simulink model "ASM_Traffic"  (R2026a)
settings: Solver=ode1  StartTime=SIM.tstart.v  StopTime=SIM.tend.v  FixedStep=SIM.StepSize.v
PostLoadFcn:
  | if any(exist('dsrtsu_mdlpostloadfcn', 'file') ~= 0), dsrtsu_mdlpostloadfcn('Execute', bdroot); end
  | try, asm_mdl_postloadfcn(bdroot, 'UpdateModel', 3600); catch, disp(lasterr); end,
InitFcn:
  | , if any(exist('rtifpga_mdlclblib', 'file') ~= 0), rtifpga_mdlclblib('Init', bdroot); end,
  | , if any(exist('dsmpb_private', 'file') ~= 0), dsmpb_private('dsmpb_mdlclblib', 'Init', bdroot); end,
model workspace (MAT data in the model file):
  asmReferencePath = [0 0.01 0.02 0.03 0.04 0.05 0.06 0.07 0.08 0.09 0.1 0.11 ... (350007 elements, 50001x7)]
  roadBounds : Simulink.Parameter (value not decoded)
  safetyAxes : Simulink.Parameter (value not decoded)
undefined symbols (not defined in the file): _to_, a0b2, ASM_BrakeHydraulics_DemoSystems, ASM_VehicleDynamics_DemoSystems, b98103fe8ad365046cd0, BrakeCircuit, controllerConfig, CPT, Crankshaft, DiscIntNeverNeededParam, dsmsi, FinalDriveAssembly, MDL, ModeSignals, mu, Pos_BrakePedal_Maneuver, rad, RefSignals, roadFamilyData, roadFamilyId, s_to_rpm, SIM, SoftECU, Suspension, Tire, Transmission
libraries: ASM_Traffic_lib x135, simulink x98, ASM_Utils_lib x77, ASM_VehicleDynamics_lib x70, ASM_Environment_lib x22, dsmpblib x20, dsmsilib x15, MDLD_Utils_lib x10, ASM_BrakeHydraulics_lib x3, sl_discontinuities x2
(part 14 of 65)

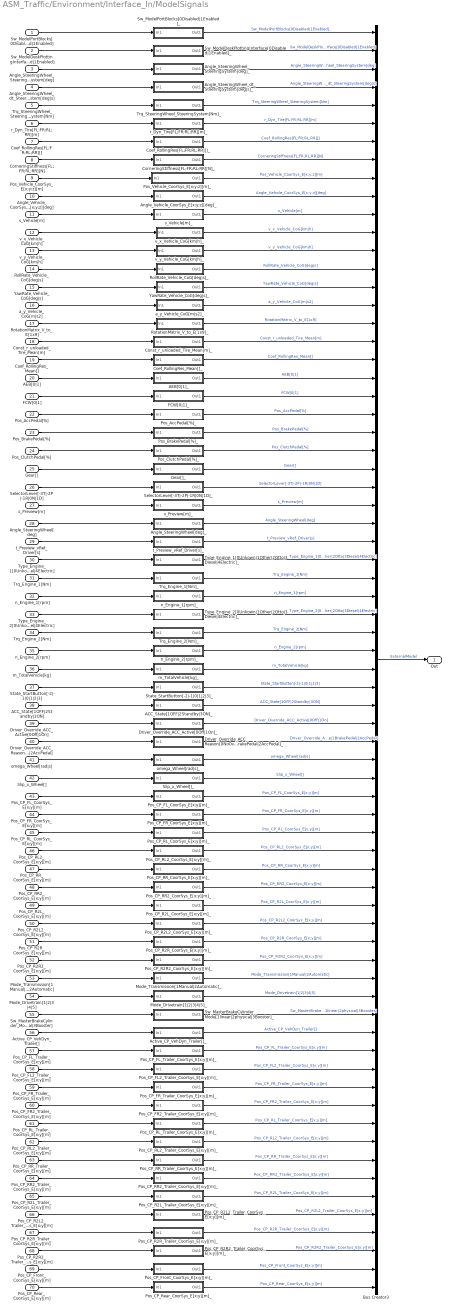
== system ASM_Traffic/Environment/Interface_In/ModelSignals ==
  Sw_ModelPortBlocks[0Disabled|1Enabled] : Inport
  Sw_ModelDeskPlottingInterface[0Disabled|1Enabled] : Inport  Port=2
  Angle_SteeringWheel_SteeringSystem[deg] : Inport  Port=3
  Angle_SteeringWheel_dt_SteeringSystem[deg|s] : Inport  Port=4
  Trq_SteeringWheel_SteeringSystem[Nm] : Inport  Port=5
  r_Dyn_Tire[FL;FR;RL;RR][m] : Inport  Port=6
  Coef_RollingRes[FL;FR;RL;RR][] : Inport  Port=7
  CorneringStiffness[FL;FR;RL;RR][N] : Inport  Port=8
  Pos_Vehicle_CoorSys_E[x;y;z][m] : Inport  Port=9
  Angle_Vehicle_CoorSys_E[x;y;z][deg] : Inport  Port=10
  s_Vehicle[m] : Inport  Port=11
  v_x_Vehicle_CoG[km|h] : Inport  Port=12
  v_y_Vehicle_CoG[km|h] : Inport  Port=13
  RollRate_Vehicle_CoG[deg|s] : Inport  Port=14
  YawRate_Vehicle_CoG[deg|s] : Inport  Port=15
  a_y_Vehicle_CoG[m|s2] : Inport  Port=16
  RotationMatrix_V_to_E[1x9] : Inport  Port=17
  Const_r_unloaded_Tire_Mean[m] : Inport  Port=18
  Coef_RollingRes_Mean[] : Inport  Port=19
  AEB[0|1] : Inport  Port=20
  FCW[0|1] : Inport  Port=21
  Pos_AccPedal[%] : Inport  Port=22
  Pos_BrakePedal[%] : Inport  Port=23
  Pos_ClutchPedal[%] : Inport  Port=24
  Gear[] : Inport  Port=25
  SelectorLever[-3T|-2P|-1R|0N|1D] : Inport  Port=26
  s_Preview[m] : Inport  Port=27
  Angle_SteeringWheel[deg] : Inport  Port=28
  t_Preview_vRef_Driver[s] : Inport  Port=29
  Type_Engine_1[0Unkown|1Other|2Otto|3Diesel|4Electric] : Inport  Port=30
  Trq_Engine_1[Nm] : Inport  Port=31
  n_Engine_1[rpm] : Inport  Port=32
  Type_Engine_2[0Unkown|1Other|2Otto|3Diesel|4Electric] : Inport  Port=33
  Trq_Engine_2[Nm] : Inport  Port=34
  n_Engine_2[rpm] : Inport  Port=35
  m_TotalVehicle[kg] : Inport  Port=36
  State_StartButton[-2|-1|0|1|2|3] : Inport  Port=37
  ACC_State[1OFF|2Standby|3ON] : Inport  Port=38
  Driver_Override_ACC_Active[0Off|1On] : Inport  Port=39
  Driver_Override_ACC_Reason[0NoOverride|1BrakePedal|2AccPedal] : Inport  Port=40
  omega_Wheel[rad|s] : Inport  Port=41
  Slip_x_Wheel[] : Inport  Port=42
  Pos_CP_FL_CoorSys_E[x;y][m] : Inport  Port=43
  Pos_CP_FR_CoorSys_E[x;y][m] : Inport  Port=44
  Pos_CP_RL_CoorSys_E[x;y][m] : Inport  Port=45
  Pos_CP_RL2_CoorSys_E[x;y][m] : Inport  Port=46
  Pos_CP_RR_CoorSys_E[x;y][m] : Inport  Port=47
  Pos_CP_RR2_CoorSys_E[x;y][m] : Inport  Port=48
  Pos_CP_R2L_CoorSys_E[x;y][m] : Inport  Port=49
  Pos_CP_R2L2_CoorSys_E[x;y][m] : Inport  Port=50
  Pos_CP_R2R_CoorSys_E[x;y][m] : Inport  Port=51
  Pos_CP_R2R2_CoorSys_E[x;y][m] : Inport  Port=52
  Mode_Transmission[1Manual|2Automatic] : Inport  Port=53
  Mode_Drivetrain[1|2|3|4|5] : Inport  Port=54
  Sw_MasterBrakeCylinder_Mode[1linear|2physical|3Booster] : Inport  Port=55
  Active_CP_VehDyn_Trailer[] : Inport  Port=56
  Pos_CP_FL_Trailer_CoorSys_E[x;y][m] : Inport  Port=57
  Pos_CP_FL2_Trailer_CoorSys_E[x;y][m] : Inport  Port=58
  Pos_CP_FR_Trailer_CoorSys_E[x;y][m] : Inport  Port=59
  Pos_CP_FR2_Trailer_CoorSys_E[x;y][m] : Inport  Port=60
  Pos_CP_RL_Trailer_CoorSys_E[x;y][m] : Inport  Port=61
  Pos_CP_RL2_Trailer_CoorSys_E[x;y][m] : Inport  Port=62
  Pos_CP_RR_Trailer_CoorSys_E[x;y][m] : Inport  Port=63
  Pos_CP_RR2_Trailer_CoorSys_E[x;y][m] : Inport  Port=64
  Pos_CP_R2L_Trailer_CoorSys_E[x;y][m] : Inport  Port=65
  Pos_CP_R2L2_Trailer_CoorSys_E[x;y][m] : Inport  Port=66
  Pos_CP_R2R_Trailer_CoorSys_E[x;y][m] : Inport  Port=67
  Pos_CP_R2R2_Trailer_CoorSys_E[x;y][m] : Inport  Port=68
  Pos_CP_Front_CoorSys_E[x;y][m] : Inport  Port=69
  Pos_CP_Rear_CoorSys_E[x;y][m] : Inport  Port=70
  ACC_State[1OFF|2Standby|3ON]_ : Subsystem
      mask Display: disp('')
  AEB[0|1]_ : Subsystem
      mask Display: disp('')
  Active_CP_VehDyn_Trailer[]_ : Subsystem
      mask Display: disp('')
  Angle_SteeringWheel[deg]_ : Subsystem
      mask Display: disp('')
  Angle_SteeringWheel_SteeringSystem[deg]_ : Subsystem
      mask Display: disp('')
  Angle_SteeringWheel_dt_SteeringSystem[deg|s]_ : Subsystem
      mask Display: disp('')
  Angle_Vehicle_CoorSys_E[x;y;z][deg]_ : Subsystem
      mask Display: disp('')
  Bus Creator3 : BusCreator  Inputs=70
  Coef_RollingRes[FL;FR;RL;RR][]_ : Subsystem
      mask Display: disp('')
  Coef_RollingRes_Mean[]_ : Subsystem
      mask Display: disp('')
  Const_r_unloaded_Tire_Mean[m]_ : Subsystem
      mask Display: disp('')
  CorneringStiffness[FL;FR;RL;RR][N]_ : Subsystem
      mask Display: disp('')
  Driver_Override_ACC_Active[0Off|1On]_ : Subsystem
      mask Display: disp('')
  Driver_Override_ACC_Reason[0NoOverride|1BrakePedal|2AccPedal]_ : Subsystem
      mask Display: disp('')
  FCW[0|1]_ : Subsystem
      mask Display: disp('')
  Gear[]_ : Subsystem
      mask Display: disp('')
  Mode_Drivetrain[1|2|3|4|5]_ : Subsystem
      mask Display: disp('')
  Mode_Transmission[1Manual|2Automatic]_ : Subsystem
      mask Display: disp('')
  Pos_AccPedal[%]_ : Subsystem
      mask Display: disp('')
  Pos_BrakePedal[%]_ : Subsystem
      mask Display: disp('')
  Pos_CP_FL2_Trailer_CoorSys_E[x;y][m]_ : Subsystem
      mask Display: disp('')
  Pos_CP_FL_CoorSys_E[x;y][m]_ : Subsystem
      mask Display: disp('')
  Pos_CP_FL_Trailer_CoorSys_E[x;y][m]_ : Subsystem
      mask Display: disp('')
  Pos_CP_FR2_Trailer_CoorSys_E[x;y][m]_ : Subsystem
      mask Display: disp('')
  Pos_CP_FR_CoorSys_E[x;y][m]_ : Subsystem
      mask Display: disp('')
  Pos_CP_FR_Trailer_CoorSys_E[x;y][m]_ : Subsystem
      mask Display: disp('')
  Pos_CP_Front_CoorSys_E[x;y][m]_ : Subsystem
      mask Display: disp('')
  Pos_CP_R2L2_CoorSys_E[x;y][m]_ : Subsystem
      mask Display: disp('')
  Pos_CP_R2L2_Trailer_CoorSys_E[x;y][m]_ : Subsystem
      mask Display: disp('')
  Pos_CP_R2L_CoorSys_E[x;y][m]_ : Subsystem
      mask Display: disp('')
  Pos_CP_R2L_Trailer_CoorSys_E[x;y][m]_ : Subsystem
      mask Display: disp('')
  Pos_CP_R2R2_CoorSys_E[x;y][m]_ : Subsystem
      mask Display: disp('')
  Pos_CP_R2R2_Trailer_CoorSys_E[x;y][m]_ : Subsystem
      mask Display: disp('')
  Pos_CP_R2R_CoorSys_E[x;y][m]_ : Subsystem
      mask Display: disp('')
  Pos_CP_R2R_Trailer_CoorSys_E[x;y][m]_ : Subsystem
      mask Display: disp('')
  Pos_CP_RL2_CoorSys_E[x;y][m]_ : Subsystem
      mask Display: disp('')
  Pos_CP_RL2_Trailer_CoorSys_E[x;y][m]_ : Subsystem
      mask Display: disp('')
  Pos_CP_RL_CoorSys_E[x;y][m]_ : Subsystem
      mask Display: disp('')
  Pos_CP_RL_Trailer_CoorSys_E[x;y][m]_ : Subsystem
      mask Display: disp('')
  Pos_CP_RR2_CoorSys_E[x;y][m]_ : Subsystem
      mask Display: disp('')
  Pos_CP_RR2_Trailer_CoorSys_E[x;y][m]_ : Subsystem
      mask Display: disp('')
  Pos_CP_RR_CoorSys_E[x;y][m]_ : Subsystem
      mask Display: disp('')
  Pos_CP_RR_Trailer_CoorSys_E[x;y][m]_ : Subsystem
      mask Display: disp('')
  Pos_CP_Rear_CoorSys_E[x;y][m]_ : Subsystem
      mask Display: disp('')
  Pos_ClutchPedal[%]_ : Subsystem
      mask Display: disp('')
  Pos_Vehicle_CoorSys_E[x;y;z][m]_ : Subsystem
      mask Display: disp('')
  RollRate_Vehicle_CoG[deg|s]_ : Subsystem
      mask Display: disp('')
  RotationMatrix_V_to_E[1x9]_ : Subsystem
      mask Display: disp('')
  SelectorLever[-3T|-2P|-1R|0N|1D]_ : Subsystem
      mask Display: disp('')
  Slip_x_Wheel[]_ : Subsystem
      mask Display: disp('')
  State_StartButton[-2|-1|0|1|2|3]_ : Subsystem
      mask Display: disp('')
  Sw_MasterBrakeCylinder_Mode[1linear|2physical|3Booster]_ : Subsystem
      mask Display: disp('')
  Sw_ModelDeskPlottingInterface[0Disabled|1Enabled]_ : Subsystem
  Sw_ModelPortBlocks[0Disabled|1Enabled]_ : Subsystem
  Trq_Engine_1[Nm]_ : Subsystem
      mask Display: disp('')
  Trq_Engine_2[Nm]_ : Subsystem
      mask Display: disp('')
  Trq_SteeringWheel_SteeringSystem[Nm]_ : Subsystem
      mask Display: disp('')
  Type_Engine_1[0Unkown|1Other|2Otto|3Diesel|4Electric]_ : Subsystem
      mask Display: disp('')
  Type_Engine_2[0Unkown|1Other|2Otto|3Diesel|4Electric]_ : Subsystem
      mask Display: disp('')
  YawRate_Vehicle_CoG[deg|s]_ : Subsystem
      mask Display: disp('')
  a_y_Vehicle_CoG[m|s2]_ : Subsystem
      mask Display: disp('')
  m_TotalVehicle[kg]_ : Subsystem
      mask Display: disp('')
  n_Engine_1[rpm]_ : Subsystem
      mask Display: disp('')
  n_Engine_2[rpm]_ : Subsystem
      mask Display: disp('')
  omega_Wheel[rad|s]_ : Subsystem
      mask Display: disp('')
  r_Dyn_Tire[FL;FR;RL;RR][m]_ : Subsystem
      mask Display: disp('')
  s_Preview[m]_ : Subsystem
      mask Display: disp('')
  s_Vehicle[m]_ : Subsystem
      mask Display: disp('')
  t_Preview_vRef_Driver[s]_ : Subsystem
      mask Display: disp('')
  v_x_Vehicle_CoG[km|h]_ : Subsystem
      mask Display: disp('')
  v_y_Vehicle_CoG[km|h]_ : Subsystem
      mask Display: disp('')
  Out : Outport  VectorParamsAs1DForOutWhenUnconnected=off
  wires:
  Pos_CP_Front_CoorSys_E[x;y][m]/1 -> Pos_CP_Front_CoorSys_E[x;y][m]_/1(In1)
  Pos_CP_Rear_CoorSys_E[x;y][m]_/1(Out1) -> Bus Creator3/70  "Pos_CP_Rear_CoorSys_E[x;y][m]"
  Pos_CP_Rear_CoorSys_E[x;y][m]/1 -> Pos_CP_Rear_CoorSys_E[x;y][m]_/1(In1)
  Pos_CP_Front_CoorSys_E[x;y][m]_/1(Out1) -> Bus Creator3/69  "Pos_CP_Front_CoorSys_E[x;y][m]"
  Sw_ModelDeskPlottingInterface[0Disabled|1Enabled]_/1(Out1) -> Bus Creator3/2  "Sw_ModelDeskPlottingInterface[0Disabled|1Enabled]"
  Sw_ModelPortBlocks[0Disabled|1Enabled]_/1(Out1) -> Bus Creator3/1  "Sw_ModelPortBlocks[0Disabled|1Enabled]"
  Sw_ModelDeskPlottingInterface[0Disabled|1Enabled]/1 -> Sw_ModelDeskPlottingInterface[0Disabled|1Enabled]_/1(In1)
  Sw_ModelPortBlocks[0Disabled|1Enabled]/1 -> Sw_ModelPortBlocks[0Disabled|1Enabled]_/1(In1)
  Bus Creator3/1 -> Out/1  "ExternalModel"
  Trq_SteeringWheel_SteeringSystem[Nm]/1 -> Trq_SteeringWheel_SteeringSystem[Nm]_/1(In1)
  Angle_SteeringWheel_SteeringSystem[deg]/1 -> Angle_SteeringWheel_SteeringSystem[deg]_/1(In1)
  Angle_SteeringWheel_SteeringSystem[deg]_/1(Out1) -> Bus Creator3/3  "Angle_SteeringWheel_SteeringSystem[deg]"
  Trq_SteeringWheel_SteeringSystem[Nm]_/1(Out1) -> Bus Creator3/5  "Trq_SteeringWheel_SteeringSystem[Nm]"
  Pos_CP_RR2_CoorSys_E[x;y][m]_/1(Out1) -> Bus Creator3/48  "Pos_CP_RR2_CoorSys_E[x;y][m]"
  Coef_RollingRes[FL;FR;RL;RR][]_/1(Out1) -> Bus Creator3/7  "Coef_RollingRes[FL;FR;RL;RR][]"
  Coef_RollingRes_Mean[]_/1(Out1) -> Bus Creator3/19  "Coef_RollingRes_Mean[]"
  Active_CP_VehDyn_Trailer[]_/1(Out1) -> Bus Creator3/56  "Active_CP_VehDyn_Trailer[]"
  Pos_CP_RR_Trailer_CoorSys_E[x;y][m]_/1(Out1) -> Bus Creator3/63  "Pos_CP_RR_Trailer_CoorSys_E[x;y][m]"
  Pos_CP_FL_Trailer_CoorSys_E[x;y][m]_/1(Out1) -> Bus Creator3/57  "Pos_CP_FL_Trailer_CoorSys_E[x;y][m]"
  Pos_CP_R2R_CoorSys_E[x;y][m]_/1(Out1) -> Bus Creator3/51  "Pos_CP_R2R_CoorSys_E[x;y][m]"
  Pos_CP_R2R2_Trailer_CoorSys_E[x;y][m]_/1(Out1) -> Bus Creator3/68  "Pos_CP_R2R2_Trailer_CoorSys_E[x;y][m]"
  Pos_CP_R2L_Trailer_CoorSys_E[x;y][m]_/1(Out1) -> Bus Creator3/65  "Pos_CP_R2L_Trailer_CoorSys_E[x;y][m]"
  Pos_CP_FR_CoorSys_E[x;y][m]_/1(Out1) -> Bus Creator3/44  "Pos_CP_FR_CoorSys_E[x;y][m]"
  Pos_CP_FR_Trailer_CoorSys_E[x;y][m]_/1(Out1) -> Bus Creator3/59  "Pos_CP_FR_Trailer_CoorSys_E[x;y][m]"
  Pos_CP_R2L2_Trailer_CoorSys_E[x;y][m]_/1(Out1) -> Bus Creator3/66  "Pos_CP_R2L2_Trailer_CoorSys_E[x;y][m]"
  Pos_CP_R2L2_CoorSys_E[x;y][m]_/1(Out1) -> Bus Creator3/50  "Pos_CP_R2L2_CoorSys_E[x;y][m]"
  Pos_CP_RL_Trailer_CoorSys_E[x;y][m]_/1(Out1) -> Bus Creator3/61  "Pos_CP_RL_Trailer_CoorSys_E[x;y][m]"
  Pos_CP_RL_CoorSys_E[x;y][m]_/1(Out1) -> Bus Creator3/45  "Pos_CP_RL_CoorSys_E[x;y][m]"
  Pos_CP_RR2_Trailer_CoorSys_E[x;y][m]_/1(Out1) -> Bus Creator3/64  "Pos_CP_RR2_Trailer_CoorSys_E[x;y][m]"
  r_Dyn_Tire[FL;FR;RL;RR][m]_/1(Out1) -> Bus Creator3/6  "r_Dyn_Tire[FL;FR;RL;RR][m]"
  Pos_CP_R2R2_CoorSys_E[x;y][m]_/1(Out1) -> Bus Creator3/52  "Pos_CP_R2R2_CoorSys_E[x;y][m]"
  Pos_CP_RR_CoorSys_E[x;y][m]_/1(Out1) -> Bus Creator3/47  "Pos_CP_RR_CoorSys_E[x;y][m]"
  Const_r_unloaded_Tire_Mean[m]_/1(Out1) -> Bus Creator3/18  "Const_r_unloaded_Tire_Mean[m]"
  Pos_CP_FR2_Trailer_CoorSys_E[x;y][m]_/1(Out1) -> Bus Creator3/60  "Pos_CP_FR2_Trailer_CoorSys_E[x;y][m]"
  Pos_CP_RL2_CoorSys_E[x;y][m]_/1(Out1) -> Bus Creator3/46  "Pos_CP_RL2_CoorSys_E[x;y][m]"
  Pos_CP_FL_CoorSys_E[x;y][m]_/1(Out1) -> Bus Creator3/43  "Pos_CP_FL_CoorSys_E[x;y][m]"
  Pos_CP_FL2_Trailer_CoorSys_E[x;y][m]_/1(Out1) -> Bus Creator3/58  "Pos_CP_FL2_Trailer_CoorSys_E[x;y][m]"
  Pos_CP_RL2_Trailer_CoorSys_E[x;y][m]_/1(Out1) -> Bus Creator3/62  "Pos_CP_RL2_Trailer_CoorSys_E[x;y][m]"
  Pos_CP_R2R_Trailer_CoorSys_E[x;y][m]_/1(Out1) -> Bus Creator3/67  "Pos_CP_R2R_Trailer_CoorSys_E[x;y][m]"
  Pos_CP_R2L_CoorSys_E[x;y][m]_/1(Out1) -> Bus Creator3/49  "Pos_CP_R2L_CoorSys_E[x;y][m]"
  CorneringStiffness[FL;FR;RL;RR][N]_/1(Out1) -> Bus Creator3/8  "CorneringStiffness[FL;FR;RL;RR][N]"
  r_Dyn_Tire[FL;FR;RL;RR][m]/1 -> r_Dyn_Tire[FL;FR;RL;RR][m]_/1(In1)
  Const_r_unloaded_Tire_Mean[m]/1 -> Const_r_unloaded_Tire_Mean[m]_/1(In1)
  Coef_RollingRes[FL;FR;RL;RR][]/1 -> Coef_RollingRes[FL;FR;RL;RR][]_/1(In1)
  Coef_RollingRes_Mean[]/1 -> Coef_RollingRes_Mean[]_/1(In1)
  CorneringStiffness[FL;FR;RL;RR][N]/1 -> CorneringStiffness[FL;FR;RL;RR][N]_/1(In1)
  Pos_CP_FL_CoorSys_E[x;y][m]/1 -> Pos_CP_FL_CoorSys_E[x;y][m]_/1(In1)
  Pos_CP_FR_CoorSys_E[x;y][m]/1 -> Pos_CP_FR_CoorSys_E[x;y][m]_/1(In1)
  Pos_CP_RL_CoorSys_E[x;y][m]/1 -> Pos_CP_RL_CoorSys_E[x;y][m]_/1(In1)
  Pos_CP_RL2_CoorSys_E[x;y][m]/1 -> Pos_CP_RL2_CoorSys_E[x;y][m]_/1(In1)
  Pos_CP_RR_CoorSys_E[x;y][m]/1 -> Pos_CP_RR_CoorSys_E[x;y][m]_/1(In1)
  Pos_CP_RR2_CoorSys_E[x;y][m]/1 -> Pos_CP_RR2_CoorSys_E[x;y][m]_/1(In1)
  Pos_CP_R2L_CoorSys_E[x;y][m]/1 -> Pos_CP_R2L_CoorSys_E[x;y][m]_/1(In1)
  Pos_CP_R2L2_CoorSys_E[x;y][m]/1 -> Pos_CP_R2L2_CoorSys_E[x;y][m]_/1(In1)
  Pos_CP_R2R_CoorSys_E[x;y][m]/1 -> Pos_CP_R2R_CoorSys_E[x;y][m]_/1(In1)
  Pos_CP_R2R2_CoorSys_E[x;y][m]/1 -> Pos_CP_R2R2_CoorSys_E[x;y][m]_/1(In1)
  Pos_CP_FL_Trailer_CoorSys_E[x;y][m]/1 -> Pos_CP_FL_Trailer_CoorSys_E[x;y][m]_/1(In1)
  Pos_CP_FL2_Trailer_CoorSys_E[x;y][m]/1 -> Pos_CP_FL2_Trailer_CoorSys_E[x;y][m]_/1(In1)
  Pos_CP_FR_Trailer_CoorSys_E[x;y][m]/1 -> Pos_CP_FR_Trailer_CoorSys_E[x;y][m]_/1(In1)
  Pos_CP_FR2_Trailer_CoorSys_E[x;y][m]/1 -> Pos_CP_FR2_Trailer_CoorSys_E[x;y][m]_/1(In1)
  Pos_CP_RL_Trailer_CoorSys_E[x;y][m]/1 -> Pos_CP_RL_Trailer_CoorSys_E[x;y][m]_/1(In1)
  Pos_CP_RL2_Trailer_CoorSys_E[x;y][m]/1 -> Pos_CP_RL2_Trailer_CoorSys_E[x;y][m]_/1(In1)
  Pos_CP_RR_Trailer_CoorSys_E[x;y][m]/1 -> Pos_CP_RR_Trailer_CoorSys_E[x;y][m]_/1(In1)
  Pos_CP_RR2_Trailer_CoorSys_E[x;y][m]/1 -> Pos_CP_RR2_Trailer_CoorSys_E[x;y][m]_/1(In1)
  Pos_CP_R2L_Trailer_CoorSys_E[x;y][m]/1 -> Pos_CP_R2L_Trailer_CoorSys_E[x;y][m]_/1(In1)
  Pos_CP_R2L2_Trailer_CoorSys_E[x;y][m]/1 -> Pos_CP_R2L2_Trailer_CoorSys_E[x;y][m]_/1(In1)
  Pos_CP_R2R_Trailer_CoorSys_E[x;y][m]/1 -> Pos_CP_R2R_Trailer_CoorSys_E[x;y][m]_/1(In1)
  Pos_CP_R2R2_Trailer_CoorSys_E[x;y][m]/1 -> Pos_CP_R2R2_Trailer_CoorSys_E[x;y][m]_/1(In1)
  Active_CP_VehDyn_Trailer[]/1 -> Active_CP_VehDyn_Trailer[]_/1(In1)
  AEB[0|1]_/1(Out1) -> Bus Creator3/20  "AEB[0|1]"
  FCW[0|1]_/1(Out1) -> Bus Creator3/21  "FCW[0|1]"
  AEB[0|1]/1 -> AEB[0|1]_/1(In1)
  FCW[0|1]/1 -> FCW[0|1]_/1(In1)
  Gear[]_/1(Out1) -> Bus Creator3/25  "Gear[]"
  s_Preview[m]_/1(Out1) -> Bus Creator3/27  "s_Preview[m]"
  Pos_ClutchPedal[%]_/1(Out1) -> Bus Creator3/24  "Pos_ClutchPedal[%]"
  SelectorLever[-3T|-2P|-1R|0N|1D]_/1(Out1) -> Bus Creator3/26  "SelectorLever[-3T|-2P|-1R|0N|1D]"
  Pos_BrakePedal[%]_/1(Out1) -> Bus Creator3/23  "Pos_BrakePedal[%]"
  t_Preview_vRef_Driver[s]_/1(Out1) -> Bus Creator3/29  "t_Preview_vRef_Driver[s]"
  Angle_SteeringWheel[deg]_/1(Out1) -> Bus Creator3/28  "Angle_SteeringWheel[deg]"
  Pos_AccPedal[%]_/1(Out1) -> Bus Creator3/22  "Pos_AccPedal[%]"
  Pos_AccPedal[%]/1 -> Pos_AccPedal[%]_/1(In1)
  Pos_BrakePedal[%]/1 -> Pos_BrakePedal[%]_/1(In1)
  Pos_ClutchPedal[%]/1 -> Pos_ClutchPedal[%]_/1(In1)
  Gear[]/1 -> Gear[]_/1(In1)
  SelectorLever[-3T|-2P|-1R|0N|1D]/1 -> SelectorLever[-3T|-2P|-1R|0N|1D]_/1(In1)
  s_Preview[m]/1 -> s_Preview[m]_/1(In1)
  Angle_SteeringWheel[deg]/1 -> Angle_SteeringWheel[deg]_/1(In1)
  t_Preview_vRef_Driver[s]/1 -> t_Preview_vRef_Driver[s]_/1(In1)
  a_y_Vehicle_CoG[m|s2]/1 -> a_y_Vehicle_CoG[m|s2]_/1(In1)
  RotationMatrix_V_to_E[1x9]_/1(Out1) -> Bus Creator3/17  "RotationMatrix_V_to_E[1x9]"
  v_x_Vehicle_CoG[km|h]/1 -> v_x_Vehicle_CoG[km|h]_/1(In1)
  Pos_Vehicle_CoorSys_E[x;y;z][m]_/1(Out1) -> Bus Creator3/9  "Pos_Vehicle_CoorSys_E[x;y;z][m]"
  v_y_Vehicle_CoG[km|h]/1 -> v_y_Vehicle_CoG[km|h]_/1(In1)
  RotationMatrix_V_to_E[1x9]/1 -> RotationMatrix_V_to_E[1x9]_/1(In1)
  Angle_Vehicle_CoorSys_E[x;y;z][deg]_/1(Out1) -> Bus Creator3/10  "Angle_Vehicle_CoorSys_E[x;y;z][deg]"
  s_Vehicle[m]_/1(Out1) -> Bus Creator3/11  "s_Vehicle[m]"
  RollRate_Vehicle_CoG[deg|s]/1 -> RollRate_Vehicle_CoG[deg|s]_/1(In1)
  YawRate_Vehicle_CoG[deg|s]_/1(Out1) -> Bus Creator3/15  "YawRate_Vehicle_CoG[deg|s]"
  RollRate_Vehicle_CoG[deg|s]_/1(Out1) -> Bus Creator3/14  "RollRate_Vehicle_CoG[deg|s]"
  s_Vehicle[m]/1 -> s_Vehicle[m]_/1(In1)
  v_y_Vehicle_CoG[km|h]_/1(Out1) -> Bus Creator3/13  "v_y_Vehicle_CoG[km|h]"
  v_x_Vehicle_CoG[km|h]_/1(Out1) -> Bus Creator3/12  "v_x_Vehicle_CoG[km|h]"
  Pos_Vehicle_CoorSys_E[x;y;z][m]/1 -> Pos_Vehicle_CoorSys_E[x;y;z][m]_/1(In1)
  a_y_Vehicle_CoG[m|s2]_/1(Out1) -> Bus Creator3/16  "a_y_Vehicle_CoG[m|s2]"
  YawRate_Vehicle_CoG[deg|s]/1 -> YawRate_Vehicle_CoG[deg|s]_/1(In1)
  Angle_Vehicle_CoorSys_E[x;y;z][deg]/1 -> Angle_Vehicle_CoorSys_E[x;y;z][deg]_/1(In1)
  Mode_Drivetrain[1|2|3|4|5]_/1(Out1) -> Bus Creator3/54  "Mode_Drivetrain[1|2|3|4|5]"
  Sw_MasterBrakeCylinder_Mode[1linear|2physical|3Booster]_/1(Out1) -> Bus Creator3/55  "Sw_MasterBrakeCylinder_Mode[1linear|2physical|3Booster]"
  Mode_Drivetrain[1|2|3|4|5]/1 -> Mode_Drivetrain[1|2|3|4|5]_/1(In1)
  Mode_Transmission[1Manual|2Automatic]_/1(Out1) -> Bus Creator3/53  "Mode_Transmission[1Manual|2Automatic]"
  Mode_Transmission[1Manual|2Automatic]/1 -> Mode_Transmission[1Manual|2Automatic]_/1(In1)
  Sw_MasterBrakeCylinder_Mode[1linear|2physical|3Booster]/1 -> Sw_MasterBrakeCylinder_Mode[1linear|2physical|3Booster]_/1(In1)
  Angle_SteeringWheel_dt_SteeringSystem[deg|s]/1 -> Angle_SteeringWheel_dt_SteeringSystem[deg|s]_/1(In1)
  Angle_SteeringWheel_dt_SteeringSystem[deg|s]_/1(Out1) -> Bus Creator3/4  "Angle_SteeringWheel_dt_SteeringSystem[deg|s]"
  n_Engine_1[rpm]/1 -> n_Engine_1[rpm]_/1(In1)
  n_Engine_1[rpm]_/1(Out1) -> Bus Creator3/32  "n_Engine_1[rpm]"
  Trq_Engine_1[Nm]_/1(Out1) -> Bus Creator3/31  "Trq_Engine_1[Nm]"
  Trq_Engine_1[Nm]/1 -> Trq_Engine_1[Nm]_/1(In1)
  m_TotalVehicle[kg]_/1(Out1) -> Bus Creator3/36  "m_TotalVehicle[kg]"
  m_TotalVehicle[kg]/1 -> m_TotalVehicle[kg]_/1(In1)
  State_StartButton[-2|-1|0|1|2|3]_/1(Out1) -> Bus Creator3/37  "State_StartButton[-2|-1|0|1|2|3]"
  State_StartButton[-2|-1|0|1|2|3]/1 -> State_StartButton[-2|-1|0|1|2|3]_/1(In1)
  ACC_State[1OFF|2Standby|3ON]_/1(Out1) -> Bus Creator3/38  "ACC_State[1OFF|2Standby|3ON]"
  ACC_State[1OFF|2Standby|3ON]/1 -> ACC_State[1OFF|2Standby|3ON]_/1(In1)
  Type_Engine_1[0Unkown|1Other|2Otto|3Diesel|4Electric]/1 -> Type_Engine_1[0Unkown|1Other|2Otto|3Diesel|4Electric]_/1(In1)
  Type_Engine_1[0Unkown|1Other|2Otto|3Diesel|4Electric]_/1(Out1) -> Bus Creator3/30  "Type_Engine_1[0Unkown|1Other|2Otto|3Diesel|4Electric]"
  Type_Engine_2[0Unkown|1Other|2Otto|3Diesel|4Electric]_/1(Out1) -> Bus Creator3/33  "Type_Engine_2[0Unkown|1Other|2Otto|3Diesel|4Electric]"
  Type_Engine_2[0Unkown|1Other|2Otto|3Diesel|4Electric]/1 -> Type_Engine_2[0Unkown|1Other|2Otto|3Diesel|4Electric]_/1(In1)
  Trq_Engine_2[Nm]/1 -> Trq_Engine_2[Nm]_/1(In1)
  Trq_Engine_2[Nm]_/1(Out1) -> Bus Creator3/34  "Trq_Engine_2[Nm]"
  n_Engine_2[rpm]_/1(Out1) -> Bus Creator3/35  "n_Engine_2[rpm]"
  n_Engine_2[rpm]/1 -> n_Engine_2[rpm]_/1(In1)
  Driver_Override_ACC_Active[0Off|1On]/1 -> Driver_Override_ACC_Active[0Off|1On]_/1(In1)
  Driver_Override_ACC_Active[0Off|1On]_/1(Out1) -> Bus Creator3/39  "Driver_Override_ACC_Active[0Off|1On]"
  Driver_Override_ACC_Reason[0NoOverride|1BrakePedal|2AccPedal]/1 -> Driver_Override_ACC_Reason[0NoOverride|1BrakePedal|2AccPedal]_/1(In1)
  Driver_Override_ACC_Reason[0NoOverride|1BrakePedal|2AccPedal]_/1(Out1) -> Bus Creator3/40  "Driver_Override_ACC_Reason[0NoOverride|1BrakePedal|2AccPedal]"
  Slip_x_Wheel[]_/1(Out1) -> Bus Creator3/42  "Slip_x_Wheel[]"
  Slip_x_Wheel[]/1 -> Slip_x_Wheel[]_/1(In1)
  omega_Wheel[rad|s]_/1(Out1) -> Bus Creator3/41  "omega_Wheel[rad|s]"
  omega_Wheel[rad|s]/1 -> omega_Wheel[rad|s]_/1(In1)

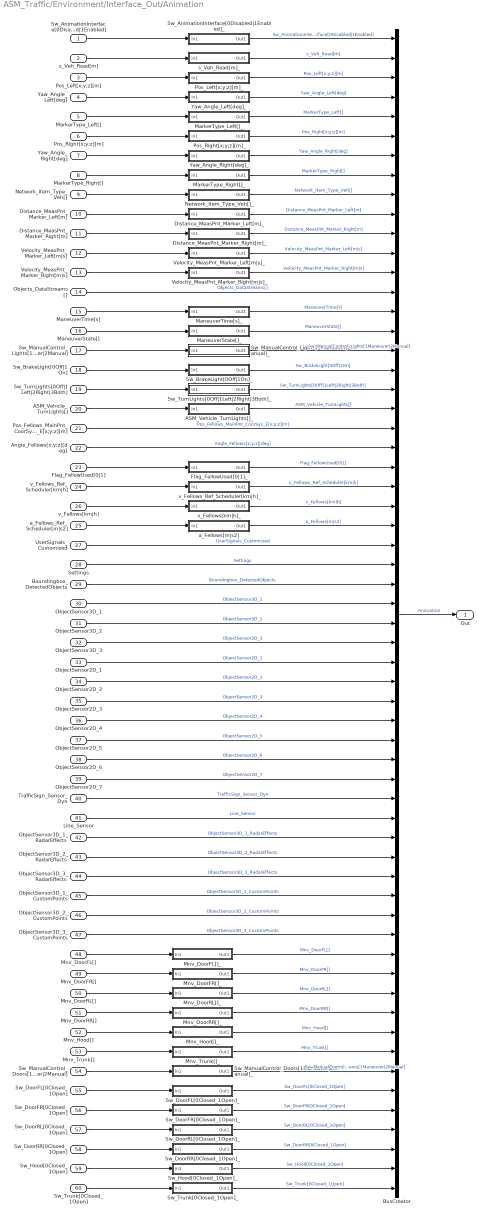
== system ASM_Traffic/Environment/Interface_Out/Animation ==
  Sw_AnimationInterface[0Disabled|1Enabled] : Inport
  s_Veh_Road[m] : Inport  Port=2
  Pos_Left[x;y;z][m] : Inport  Port=3
  Yaw_Angle_Left[deg] : Inport  Port=4
  MarkerType_Left[] : Inport  Port=5
  Pos_Right[x;y;z][m] : Inport  Port=6
  Yaw_Angle_Right[deg] : Inport  Port=7
  MarkerType_Right[] : Inport  Port=8
  Network_Item_Type_Veh[] : Inport  Port=9
  Distance_MeasPnt_Marker_Left[m] : Inport  Port=10
  Distance_MeasPnt_Marker_Right[m] : Inport  Port=11
  Velocity_MeasPnt_Marker_Left[m|s] : Inport  Port=12
  Velocity_MeasPnt_Marker_Right[m|s] : Inport  Port=13
  Objects_DataStreams[] : Inport  Port=14
  ManeuverTime[s] : Inport  Port=15
  ManeuverState[] : Inport  Port=16
  Sw_ManualControl_Lights[1Maneuver|2Manual] : Inport  Port=17
  Sw_BrakeLight[0Off|1On] : Inport  Port=18
  Sw_TurnLights[0Off|1Left|2Right|3Both] : Inport  Port=19
  ASM_Vehicle_TurnLights[] : Inport  Port=20
  Pos_Fellows_MainPnt_CoorSys_E[x;y;z][m] : Inport  Port=21
  Angle_Fellows[x;y;z][deg] : Inport  Port=22
  Flag_FellowUsed[0|1] : Inport  Port=23
  v_Fellows_Ref_Scheduler[km|h] : Inport  Port=24
  a_Fellows_Ref_Scheduler[m|s2] : Inport  Port=25
  v_Fellows[km|h] : Inport  Port=26
  UserSignals_Customized : Inport  Port=27
  Settings : Inport  Port=28
  Boundingbox_DetectedObjects : Inport  Port=29
  ObjectSensor3D_1 : Inport  Port=30
  ObjectSensor3D_2 : Inport  Port=31
  ObjectSensor3D_3 : Inport  Port=32
  ObjectSensor2D_1 : Inport  Port=33
  ObjectSensor2D_2 : Inport  Port=34
  ObjectSensor2D_3 : Inport  Port=35
  ObjectSensor2D_4 : Inport  Port=36
  ObjectSensor2D_5 : Inport  Port=37
  ObjectSensor2D_6 : Inport  Port=38
  ObjectSensor2D_7 : Inport  Port=39
  TrafficSign_Sensor_Dyn : Inport  Port=40
  Line_Sensor : Inport  Port=41
  ObjectSensor3D_1_RadarEffects : Inport  Port=42
  ObjectSensor3D_2_RadarEffects : Inport  Port=43
  ObjectSensor3D_3_RadarEffects : Inport  Port=44
  ObjectSensor3D_1_CustomPoints : Inport  Port=45
  ObjectSensor3D_2_CustomPoints : Inport  Port=46
  ObjectSensor3D_3_CustomPoints : Inport  Port=47
  Mnv_DoorFL[] : Inport  Port=48
  Mnv_DoorFR[] : Inport  Port=49
  Mnv_DoorRL[] : Inport  Port=50
  Mnv_DoorRR[] : Inport  Port=51
  Mnv_Hood[] : Inport  Port=52
  Mnv_Trunk[] : Inport  Port=53
  Sw_ManualControl_Doors[1Maneuver|2Manual] : Inport  Port=54
  Sw_DoorFL[0Closed_1Open] : Inport  Port=55
  Sw_DoorFR[0Closed_1Open] : Inport  Port=56
  Sw_DoorRL[0Closed_1Open] : Inport  Port=57
  Sw_DoorRR[0Closed_1Open] : Inport  Port=58
  Sw_Hood[0Closed_1Open] : Inport  Port=59
  Sw_Trunk[0Closed_1Open] : Inport  Port=60
  ASM_Vehicle_TurnLights[]_ : Subsystem
      mask Display: disp('')
  BusCreator : BusCreator  Inputs=60
  Distance_MeasPnt_Marker_Left[m]_ : Subsystem
      mask Display: disp('')
  Distance_MeasPnt_Marker_Right[m]_ : Subsystem
      mask Display: disp('')
  Flag_FellowUsed[0|1]_ : Subsystem
      mask Display: disp('')
  ManeuverState[]_ : Subsystem
      mask Display: disp('')
  ManeuverTime[s]_ : Subsystem
      mask Display: disp('')
  MarkerType_Left[]_ : Subsystem
      mask Display: disp('')
  MarkerType_Right[]_ : Subsystem
      mask Display: disp('')
  Mnv_DoorFL[]_ : Subsystem
      mask Display: disp('')
  Mnv_DoorFR[]_ : Subsystem
      mask Display: disp('')
  Mnv_DoorRL[]_ : Subsystem
      mask Display: disp('')
  Mnv_DoorRR[]_ : Subsystem
      mask Display: disp('')
  Mnv_Hood[]_ : Subsystem
      mask Display: disp('')
  Mnv_Trunk[]_ : Subsystem
      mask Display: disp('')
  Network_Item_Type_Veh[]_ : Subsystem
      mask Display: disp('')
  Pos_Left[x;y;z][m]_ : Subsystem
      mask Display: disp('')
  Pos_Right[x;y;z][m]_ : Subsystem
      mask Display: disp('')
  Sw_AnimationInterface[0Disabled|1Enabled]_ : Subsystem
      mask Display: disp('')
  Sw_BrakeLight[0Off|1On]_ : Subsystem
      mask Display: disp('')
  Sw_DoorFL[0Closed_1Open]_ : Subsystem
      mask Display: disp('')
  Sw_DoorFR[0Closed_1Open]_ : Subsystem
      mask Display: disp('')
  Sw_DoorRL[0Closed_1Open]_ : Subsystem
      mask Display: disp('')
  Sw_DoorRR[0Closed_1Open]_ : Subsystem
      mask Display: disp('')
  Sw_Hood[0Closed_1Open]_ : Subsystem
      mask Display: disp('')
  Sw_ManualControl_Doors[1Maneuver|2Manual]_ : Subsystem
      mask Display: disp('')
  Sw_ManualControl_Lights[1Maneuver|2Manual]_ : Subsystem
      mask Display: disp('')
  Sw_Trunk[0Closed_1Open]_ : Subsystem
      mask Display: disp('')
  Sw_TurnLights[0Off|1Left|2Right|3Both]_ : Subsystem
      mask Display: disp('')
  Velocity_MeasPnt_Marker_Left[m|s]_ : Subsystem
      mask Display: disp('')
  Velocity_MeasPnt_Marker_Right[m|s]_ : Subsystem
      mask Display: disp('')
  Yaw_Angle_Left[deg]_ : Subsystem
      mask Display: disp('')
  Yaw_Angle_Right[deg]_ : Subsystem
      mask Display: disp('')
  a_Fellows[m|s2] : Subsystem
      mask Display: disp('')
  s_Veh_Road[m]_ : Subsystem
      mask Display: disp('')
  v_Fellows[km|h]_ : Subsystem
      mask Display: disp('')
  v_Fellows_Ref_Scheduler[km|h]_ : Subsystem
      mask Display: disp('')
  Out : Outport  VectorParamsAs1DForOutWhenUnconnected=off
  wires:
  Sw_AnimationInterface[0Disabled|1Enabled]_/1(Out1) -> BusCreator/1  "Sw_AnimationInterface[0Disabled|1Enabled]"
  Sw_AnimationInterface[0Disabled|1Enabled]/1 -> Sw_AnimationInterface[0Disabled|1Enabled]_/1(In1)
  a_Fellows[m|s2]/1(Out1) -> BusCreator/26  "a_Fellows[m|s2]"
  a_Fellows_Ref_Scheduler[m|s2]/1 -> a_Fellows[m|s2]/1(In1)
  ObjectSensor2D_1/1 -> BusCreator/33  "ObjectSensor2D_1"
  ObjectSensor2D_2/1 -> BusCreator/34  "ObjectSensor2D_2"
  ObjectSensor3D_1/1 -> BusCreator/30  "ObjectSensor3D_1"
  ObjectSensor2D_3/1 -> BusCreator/35  "ObjectSensor2D_3"
  ObjectSensor3D_2/1 -> BusCreator/31  "ObjectSensor3D_2"
  ObjectSensor2D_6/1 -> BusCreator/38  "ObjectSensor2D_6"
  ObjectSensor2D_4/1 -> BusCreator/36  "ObjectSensor2D_4"
  ObjectSensor2D_7/1 -> BusCreator/39  "ObjectSensor2D_7"
  TrafficSign_Sensor_Dyn/1 -> BusCreator/40  "TrafficSign_Sensor_Dyn"
  ObjectSensor3D_3_CustomPoints/1 -> BusCreator/47  "ObjectSensor3D_3_CustomPoints"
  ObjectSensor3D_3/1 -> BusCreator/32  "ObjectSensor3D_3"
  ObjectSensor3D_1_RadarEffects/1 -> BusCreator/42  "ObjectSensor3D_1_RadarEffects"
  ObjectSensor3D_3_RadarEffects/1 -> BusCreator/44  "ObjectSensor3D_3_RadarEffects"
  ObjectSensor3D_2_CustomPoints/1 -> BusCreator/46  "ObjectSensor3D_2_CustomPoints"
  ObjectSensor2D_5/1 -> BusCreator/37  "ObjectSensor2D_5"
  Line_Sensor/1 -> BusCreator/41  "Line_Sensor"
  ObjectSensor3D_1_CustomPoints/1 -> BusCreator/45  "ObjectSensor3D_1_CustomPoints"
  ObjectSensor3D_2_RadarEffects/1 -> BusCreator/43  "ObjectSensor3D_2_RadarEffects"
  Boundingbox_DetectedObjects/1 -> BusCreator/29  "Boundingbox_DetectedObjects"
  v_Fellows[km|h]_/1(Out1) -> BusCreator/25  "v_Fellows[km|h]"
  v_Fellows_Ref_Scheduler[km|h]_/1(Out1) -> BusCreator/24  "v_Fellows_Ref_Scheduler[km|h]"
  Flag_FellowUsed[0|1]_/1(Out1) -> BusCreator/23  "Flag_FellowUsed[0|1]"
  Pos_Fellows_MainPnt_CoorSys_E[x;y;z][m]/1 -> BusCreator/21  "Pos_Fellows_MainPnt_CoorSys_E[x;y;z][m]"
  Settings/1 -> BusCreator/28  "Settings"
  v_Fellows_Ref_Scheduler[km|h]/1 -> v_Fellows_Ref_Scheduler[km|h]_/1(In1)
  UserSignals_Customized/1 -> BusCreator/27  "UserSignals_Customized"
  Angle_Fellows[x;y;z][deg]/1 -> BusCreator/22  "Angle_Fellows[x;y;z][deg]"
  v_Fellows[km|h]/1 -> v_Fellows[km|h]_/1(In1)
  Flag_FellowUsed[0|1]/1 -> Flag_FellowUsed[0|1]_/1(In1)
  ASM_Vehicle_TurnLights[]_/1(Out1) -> BusCreator/20  "ASM_Vehicle_TurnLights[]"
  Sw_TurnLights[0Off|1Left|2Right|3Both]_/1(Out1) -> BusCreator/19  "Sw_TurnLights[0Off|1Left|2Right|3Both]"
  Sw_BrakeLight[0Off|1On]_/1(Out1) -> BusCreator/18  "Sw_BrakeLight[0Off|1On]"
  Sw_ManualControl_Lights[1Maneuver|2Manual]_/1(Out1) -> BusCreator/17  "Sw_ManualControl_Lights[1Maneuver|2Manual]"
  ManeuverState[]_/1(Out1) -> BusCreator/16  "ManeuverState[]"
  ManeuverTime[s]_/1(Out1) -> BusCreator/15  "ManeuverTime[s]"
  ManeuverState[]/1 -> ManeuverState[]_/1(In1)
  Sw_BrakeLight[0Off|1On]/1 -> Sw_BrakeLight[0Off|1On]_/1(In1)
  ManeuverTime[s]/1 -> ManeuverTime[s]_/1(In1)
  Sw_TurnLights[0Off|1Left|2Right|3Both]/1 -> Sw_TurnLights[0Off|1Left|2Right|3Both]_/1(In1)
  Sw_ManualControl_Lights[1Maneuver|2Manual]/1 -> Sw_ManualControl_Lights[1Maneuver|2Manual]_/1(In1)
  ASM_Vehicle_TurnLights[]/1 -> ASM_Vehicle_TurnLights[]_/1(In1)
  Objects_DataStreams[]/1 -> BusCreator/14  "Objects_DataStreams[]"
  Velocity_MeasPnt_Marker_Right[m|s]_/1(Out1) -> BusCreator/13  "Velocity_MeasPnt_Marker_Right[m|s]"
  Velocity_MeasPnt_Marker_Left[m|s]_/1(Out1) -> BusCreator/12  "Velocity_MeasPnt_Marker_Left[m|s]"
  Distance_MeasPnt_Marker_Right[m]_/1(Out1) -> BusCreator/11  "Distance_MeasPnt_Marker_Right[m]"
  Distance_MeasPnt_Marker_Left[m]_/1(Out1) -> BusCreator/10  "Distance_MeasPnt_Marker_Left[m]"
  Network_Item_Type_Veh[]_/1(Out1) -> BusCreator/9  "Network_Item_Type_Veh[]"
  MarkerType_Right[]_/1(Out1) -> BusCreator/8  "MarkerType_Right[]"
  Yaw_Angle_Right[deg]_/1(Out1) -> BusCreator/7  "Yaw_Angle_Right[deg]"
  Pos_Right[x;y;z][m]_/1(Out1) -> BusCreator/6  "Pos_Right[x;y;z][m]"
  MarkerType_Left[]_/1(Out1) -> BusCreator/5  "MarkerType_Left[]"
  Yaw_Angle_Left[deg]_/1(Out1) -> BusCreator/4  "Yaw_Angle_Left[deg]"
  Pos_Left[x;y;z][m]_/1(Out1) -> BusCreator/3  "Pos_Left[x;y;z][m]"
  s_Veh_Road[m]_/1(Out1) -> BusCreator/2  "s_Veh_Road[m]"
  s_Veh_Road[m]/1 -> s_Veh_Road[m]_/1(In1)
  Pos_Left[x;y;z][m]/1 -> Pos_Left[x;y;z][m]_/1(In1)
  Pos_Right[x;y;z][m]/1 -> Pos_Right[x;y;z][m]_/1(In1)
  Yaw_Angle_Left[deg]/1 -> Yaw_Angle_Left[deg]_/1(In1)
  Distance_MeasPnt_Marker_Right[m]/1 -> Distance_MeasPnt_Marker_Right[m]_/1(In1)
  MarkerType_Left[]/1 -> MarkerType_Left[]_/1(In1)
  MarkerType_Right[]/1 -> MarkerType_Right[]_/1(In1)
  Yaw_Angle_Right[deg]/1 -> Yaw_Angle_Right[deg]_/1(In1)
  Velocity_MeasPnt_Marker_Right[m|s]/1 -> Velocity_MeasPnt_Marker_Right[m|s]_/1(In1)
  Network_Item_Type_Veh[]/1 -> Network_Item_Type_Veh[]_/1(In1)
  Velocity_MeasPnt_Marker_Left[m|s]/1 -> Velocity_MeasPnt_Marker_Left[m|s]_/1(In1)
  Distance_MeasPnt_Marker_Left[m]/1 -> Distance_MeasPnt_Marker_Left[m]_/1(In1)
  BusCreator/1 -> Out/1  "Animation"
  Mnv_Trunk[]/1 -> Mnv_Trunk[]_/1(In1)
  Mnv_DoorFR[]/1 -> Mnv_DoorFR[]_/1(In1)
  Mnv_Hood[]/1 -> Mnv_Hood[]_/1(In1)
  Mnv_DoorRL[]/1 -> Mnv_DoorRL[]_/1(In1)
  Mnv_DoorRR[]/1 -> Mnv_DoorRR[]_/1(In1)
  Mnv_DoorFL[]_/1(Out1) -> BusCreator/48  "Mnv_DoorFL[]"
  Mnv_DoorFL[]/1 -> Mnv_DoorFL[]_/1(In1)
  Mnv_DoorFR[]_/1(Out1) -> BusCreator/49  "Mnv_DoorFR[]"
  Mnv_DoorRL[]_/1(Out1) -> BusCreator/50  "Mnv_DoorRL[]"
  Mnv_DoorRR[]_/1(Out1) -> BusCreator/51  "Mnv_DoorRR[]"
  Mnv_Hood[]_/1(Out1) -> BusCreator/52  "Mnv_Hood[]"
  Mnv_Trunk[]_/1(Out1) -> BusCreator/53  "Mnv_Trunk[]"
  Sw_DoorFL[0Closed_1Open]_/1(Out1) -> BusCreator/55  "Sw_DoorFL[0Closed_1Open]"
  Sw_DoorFR[0Closed_1Open]_/1(Out1) -> BusCreator/56  "Sw_DoorFR[0Closed_1Open]"
  Sw_ManualControl_Doors[1Maneuver|2Manual]_/1(Out1) -> BusCreator/54  "Sw_ManualControl_Doors[1Maneuver|2Manual]"
  Sw_Hood[0Closed_1Open]_/1(Out1) -> BusCreator/59  "Sw_Hood[0Closed_1Open]"
  Sw_DoorRR[0Closed_1Open]_/1(Out1) -> BusCreator/58  "Sw_DoorRR[0Closed_1Open]"
  Sw_DoorRL[0Closed_1Open]_/1(Out1) -> BusCreator/57  "Sw_DoorRL[0Closed_1Open]"
  Sw_Trunk[0Closed_1Open]_/1(Out1) -> BusCreator/60  "Sw_Trunk[0Closed_1Open]"
  Sw_ManualControl_Doors[1Maneuver|2Manual]/1 -> Sw_ManualControl_Doors[1Maneuver|2Manual]_/1(In1)
  Sw_DoorFL[0Closed_1Open]/1 -> Sw_DoorFL[0Closed_1Open]_/1(In1)
  Sw_DoorFR[0Closed_1Open]/1 -> Sw_DoorFR[0Closed_1Open]_/1(In1)
  Sw_DoorRL[0Closed_1Open]/1 -> Sw_DoorRL[0Closed_1Open]_/1(In1)
  Sw_DoorRR[0Closed_1Open]/1 -> Sw_DoorRR[0Closed_1Open]_/1(In1)
  Sw_Hood[0Closed_1Open]/1 -> Sw_Hood[0Closed_1Open]_/1(In1)
  Sw_Trunk[0Closed_1Open]/1 -> Sw_Trunk[0Closed_1Open]_/1(In1)
